simulink model "furuta_harness"  (R2026a)
settings: Solver=ode4  StopTime=hT  FixedStep=hcfg.dt
PostLoadFcn:
  | addpath(fileparts(get_param('furuta_harness', 'FileName')));
  | harness_load('LqrBalance', 'balance', 'IfMissing', true, 'Open', false);
values from neighbouring files (symbols this model uses):
  hp = V.hp    [run_sim.m]
  m = R.metrics    [compare_controllers.m]
  N = round(opts.T/h)    [validate_open_loop.m]
  s = names{code + 1}    [run_sim.m]
  X = xn(n, :)'    [validate_open_loop.m]
undefined symbols (not defined in the file or in its folder): ctrlP, hb, hcfg, hx0, Y, Z
libraries: sm_lib x13, nesl_utility x7
settings Model: Creator=ahmad  LastModifiedBy=ahmad
settings DebuggingCC: AlgebraicLoopMsg=error
settings ExplorerConfigSet: SimMechanicsOpenEditorOnUpdate=off

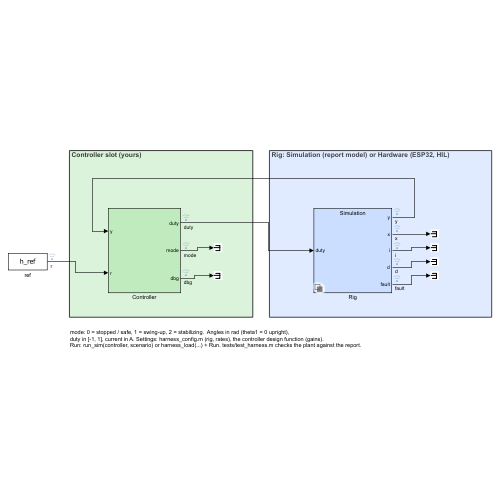
[thumbnail: Simulink's stored preview of the top-level diagram]
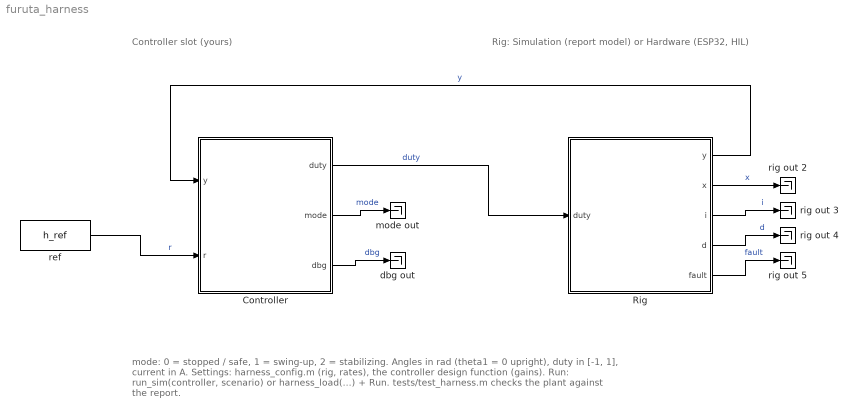
== system furuta_harness ==
  note: Controller slot (yours)
  note: Rig: Simulation (report model) or Hardware (ESP32, HIL)
  note: mode: 0 = stopped / safe, 1 = swing-up, 2 = stabilizing.  Angles in rad (theta1 = 0 upright),
      | duty in [-1, 1], current in A. Settings: harness_config.m (rig, rates), the controller design function (gains).
      | Run: run_sim(controller, scenario) or harness_load(...) + Run. tests/test_harness.m checks the plant against the report.
  Controller : Subsystem
  Rig : Subsystem  Variant=on  VariantControlMode=label  LabelModeActiveChoice=Simulation
  dbg out : Terminator
  mode out : Terminator
  ref : FromWorkspace  VariableName=h_ref  SampleTime=hcfg.Ts  Interpolate=off  OutputAfterFinalValue=Holding final value
  rig out {2..5} (4 alike) : Terminator
  wires:
  ref/1 -> Controller/2(r)  "r"
  Controller/1(duty) -> Rig/1(duty)  "duty"
  Controller/2(mode) -> mode out/1  "mode"
  Controller/3(dbg) -> dbg out/1  "dbg"
  Rig/2(x) -> rig out 2/1  "x"
  Rig/3(i) -> rig out 3/1  "i"
  Rig/4(d) -> rig out 4/1  "d"
  Rig/5(fault) -> rig out 5/1  "fault"
  Rig/1(y) -> Controller/1(y)  "y"

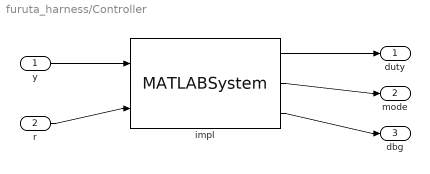
== system furuta_harness/Controller ==
  y : Inport
  r : Inport  Port=2
  impl : MATLABSystem  System=LqrBalance  Ts=hcfg.Ts  P=ctrlP  SimulateUsing=Interpreted execution
      mask Type: LqrBalance
  duty : Outport
  mode : Outport  Port=2
  dbg : Outport  Port=3
  wires:
  y/1 -> impl/1
  r/1 -> impl/2
  impl/1 -> duty/1
  impl/2 -> mode/1
  impl/3 -> dbg/1

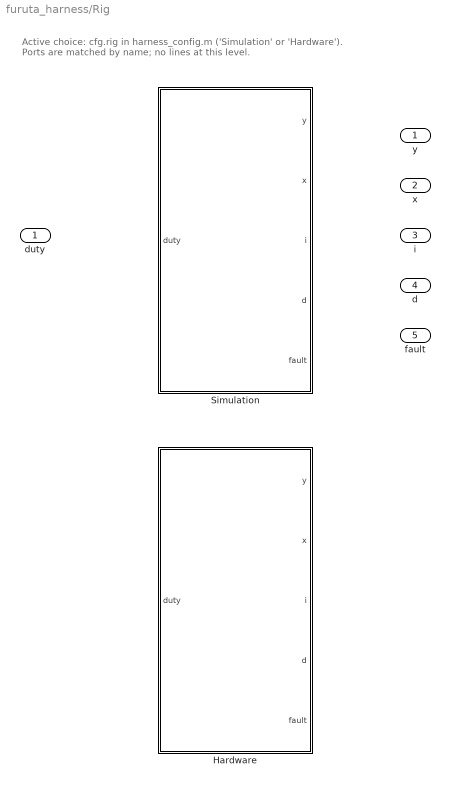
== system furuta_harness/Rig ==
  note: Active choice: cfg.rig in harness_config.m ('Simulation' or 'Hardware').
      | Ports are matched by name; no lines at this level.
  duty : Inport
  Hardware : Subsystem  VariantControl=Hardware
  Simulation : Subsystem  VariantControl=Simulation
  y : Outport
  x : Outport  Port=2
  i : Outport  Port=3
  d : Outport  Port=4
  fault : Outport  Port=5

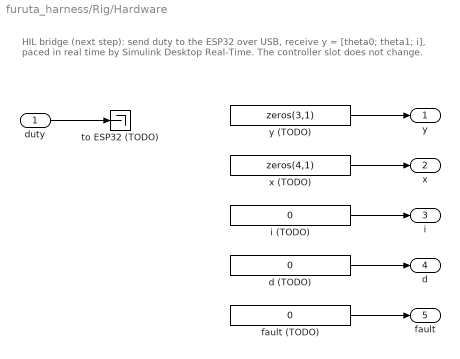
== system furuta_harness/Rig/Hardware ==
  note: HIL bridge (next step): send duty to the ESP32 over USB, receive y = [theta0; theta1; i],
      | paced in real time by Simulink Desktop Real-Time. The controller slot does not change.
  duty : Inport
  d (TODO) : Constant  Value=0  SampleTime=hcfg.Ts
  fault (TODO) : Constant  Value=0  SampleTime=hcfg.Ts
  i (TODO) : Constant  Value=0  SampleTime=hcfg.Ts
  to ESP32 (TODO) : Terminator
  x (TODO) : Constant  Value=zeros(4,1)  SampleTime=hcfg.Ts
  y (TODO) : Constant  Value=zeros(3,1)  SampleTime=hcfg.Ts
  y : Outport
  x : Outport  Port=2
  i : Outport  Port=3
  d : Outport  Port=4
  fault : Outport  Port=5
  wires:
  duty/1 -> to ESP32 (TODO)/1
  y (TODO)/1 -> y/1
  x (TODO)/1 -> x/1
  i (TODO)/1 -> i/1
  d (TODO)/1 -> d/1
  fault (TODO)/1 -> fault/1

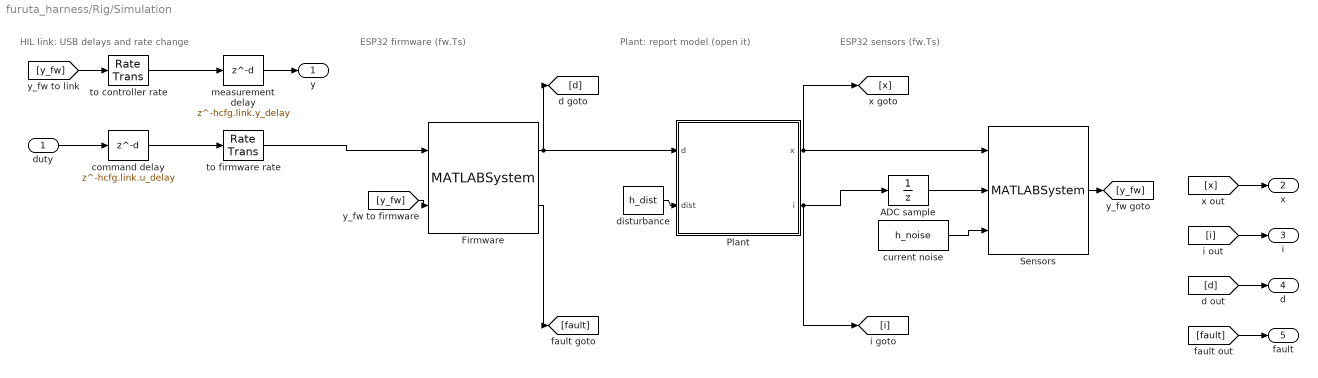
== system furuta_harness/Rig/Simulation ==
  note: HIL link: USB delays and rate change
  note: ESP32 firmware (fw.Ts)
  note: Plant: report model (open it)
  note: ESP32 sensors (fw.Ts)
  duty : Inport
  ADC sample : UnitDelay  SampleTime=hcfg.fw.Ts
  Firmware : MATLABSystem  System=FirmwareActuator  Ts=hcfg.fw.Ts  A=hcfg.act  SimulateUsing=Interpreted execution
      mask Type: FirmwareActuator
  Plant : Subsystem
  Sensors : MATLABSystem  System=FurutaSensors  Ts=hcfg.fw.Ts  S=hcfg.sens  SimulateUsing=Interpreted execution
      mask Type: FurutaSensors
  command delay : Delay  DelayLength=hcfg.link.u_delay  SampleTime=hcfg.Ts
  current noise : FromWorkspace  VariableName=h_noise  SampleTime=hcfg.fw.Ts  Interpolate=off  OutputAfterFinalValue=Holding final value
  disturbance : FromWorkspace  VariableName=h_dist  SampleTime=hcfg.dt  Interpolate=off  OutputAfterFinalValue=Holding final value
  measurement delay : Delay  DelayLength=hcfg.link.y_delay  SampleTime=hcfg.Ts
  to controller rate : RateTransition  Integrity=off  Deterministic=off  OutPortSampleTime=hcfg.Ts
  to firmware rate : RateTransition  Integrity=off  Deterministic=off  OutPortSampleTime=hcfg.fw.Ts
  y : Outport
  x : Outport  Port=2
  i : Outport  Port=3
  d : Outport  Port=4
  fault : Outport  Port=5
  wires:
  [y_fw] -> to controller rate/1
  to controller rate/1 -> measurement delay/1
  measurement delay/1 -> y/1
  duty/1 -> command delay/1
  command delay/1 -> to firmware rate/1
  to firmware rate/1 -> Firmware/1
  [y_fw] -> Firmware/2
  Firmware/2 -> [fault]
  Firmware/1 -> Plant/1(d), [d]
  disturbance/1 -> Plant/2(dist)
  Plant/1(x) -> Sensors/1, [x]
  Plant/2(i) -> ADC sample/1, [i]
  ADC sample/1 -> Sensors/2
  current noise/1 -> Sensors/3
  Sensors/1 -> [y_fw]
  [x] -> x/1
  [i] -> i/1
  [d] -> d/1
  [fault] -> fault/1

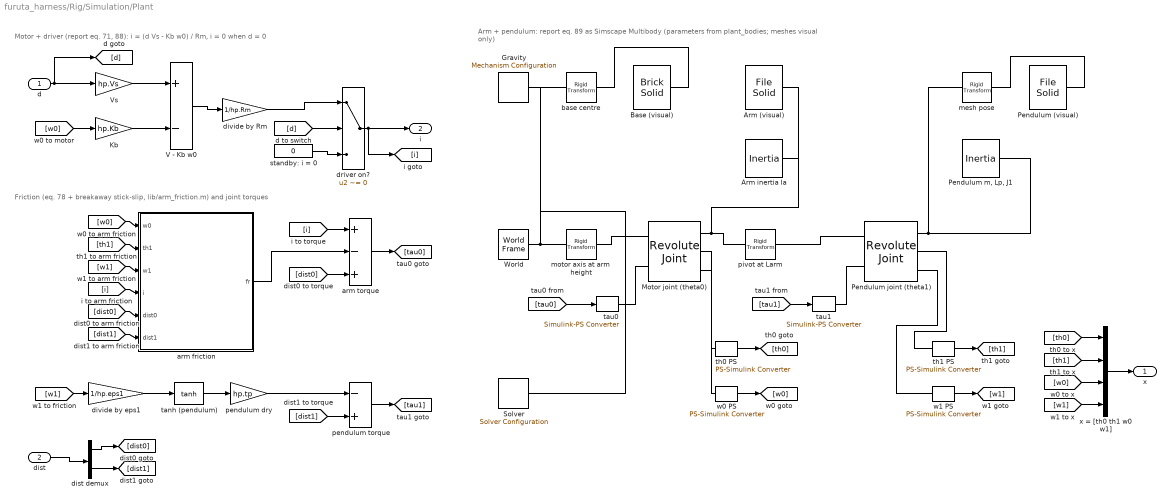
== system furuta_harness/Rig/Simulation/Plant ==
  note: Motor + driver (report eq. 71, 88): i = (d Vs - Kb w0) / Rm, i = 0 when d = 0
  note: Friction (eq. 78 + breakaway stick-slip, lib/arm_friction.m) and joint torques
  note: Arm + pendulum: report eq. 89 as Simscape Multibody (parameters from plant_bodies; meshes visual only)
  d : Inport
  dist : Inport  Port=2
  Arm (visual) : sm_lib/Body Elements/File Solid  ExtGeomFileName=body_arm_jumper3.stl  UnitType=Custom  ExtGeomFileUnits=mm  StepReaderType=HEX  ExportConvexHullGeometry=off  InertiaType=PointMass  BasedOnType=DensityFromFile  Density=1000  DensityUnits=kg/m^3  Mass=1e-9  MassUnits=kg  CenterOfMass=[0 0 0]  CenterOfMassUnits=m  MomentsOfInertia=[1 1 1]  MomentsOfInertiaUnits=kg*m^2  ProductsOfInertia=[0 0 0]  ProductsOfInertiaUnits=kg*m^2  GraphicType=FromGeometry  MarkerShape=Sphere  MarkerSize=10  GraphicVisPropType=SimpleVisualProperties  GraphicDiffuseColor=[0.15 0.15 0.17]  GraphicOpacity=1  GraphicSpecularColor=[0.5 0.5 0.5 1.0]  GraphicAmbientColor=[0.15 0.15 0.15 1.0]  GraphicEmissiveColor=[0.0 0.0 0.0 1.0]  GraphicShininess=75  DoExposeReferenceFrame=on  SerializedFrames=<Frames/>
  Arm inertia Ia : sm_lib/Body Elements/Inertia  InertiaType=Custom  Mass=hb.m_arm  MassUnits=kg  CenterOfMass=[0 0 0]  CenterOfMassUnits=m  MomentsOfInertia=[hb.Ia/2 hb.Ia/2 hb.Ia]  MomentsOfInertiaUnits=kg*m^2  ProductsOfInertia=[0 0 0]  ProductsOfInertiaUnits=kg*m^2  GraphicType=Marker  MarkerShape=Inertia  MarkerSize=20  GraphicVisPropType=SimpleVisualProperties  GraphicDiffuseColor=[0.5 0.5 0.5]  GraphicOpacity=1  GraphicSpecularColor=[0.5 0.5 0.5 1.0]  GraphicAmbientColor=[0.15 0.15 0.15 1.0]  GraphicEmissiveColor=[0.0 0.0 0.0 1.0]  GraphicShininess=75
  Base (visual) : sm_lib/Body Elements/Brick Solid  BrickDimensions=[0.0872 0.0872 0.1]  BrickDimensionsUnits=m  ExportEntireGeometry=off  InertiaType=PointMass  BasedOnType=Density  Density=1000  DensityUnits=kg/m^3  Mass=1e-9  MassUnits=kg  CenterOfMass=[0 0 0]  CenterOfMassUnits=m  MomentsOfInertia=[1 1 1]  MomentsOfInertiaUnits=kg*m^2  ProductsOfInertia=[0 0 0]  ProductsOfInertiaUnits=kg*m^2  GraphicType=FromGeometry  MarkerShape=Sphere  MarkerSize=10  GraphicVisPropType=SimpleVisualProperties  GraphicDiffuseColor=[0.6 0.62 0.65]  GraphicOpacity=0.4  GraphicSpecularColor=[0.5 0.5 0.5 1.0]  GraphicAmbientColor=[0.15 0.15 0.15 1.0]  GraphicEmissiveColor=[0.0 0.0 0.0 1.0]  GraphicShininess=75  DoExposeReferenceFrame=on  SerializedFrames=<Frames/>
  Gravity : sm_lib/Utilities/Mechanism Configuration  UniformGravity=Constant  GravityVector=[0 0 -hb.g]  GravityVectorUnits=m/s^2  LinearizationDelta=0.001  JointModeTransitionNonlinearIterations=2
  Kb : Gain  Gain=hp.Kb
  Motor joint (theta0) : sm_lib/Joints/Revolute Joint  JointMode=Normal  CompositeWrenchDir=FollowerOnBase  CompositeWrenchFrame=BaseFrame  SenseConstraintForce=off  SenseConstraintTorque=off  SenseTotalForce=off  SenseTotalTorque=off  PositionTargetSpecify=on  PositionTargetPriority=High  PositionTargetValue=hx0(1)  PositionTargetValueUnits=rad  VelocityTargetSpecify=on  VelocityTargetPriority=High  VelocityTargetValue=hx0(3)  VelocityTargetValueUnits=rad/s  EquilibriumPosition=0  EquilibriumPositionUnits=deg  SpringStiffness=0  SpringStiffnessUnits=N*m/deg  DampingCoefficient=hp.Beq  DampingCoefficientUnits=N*m/(rad/s)  LowerLimitSpecify=off  LowerLimitBound=-90  LowerLimitBoundUnits=deg  LowerLimitStiffness=1e4  LowerLimitStiffnessUnits=N*m/deg  LowerLimitDamping=10  LowerLimitDampingUnits=N*m/(deg/s)  LowerLimitTransitionRegionWidth=0.1  LowerLimitTransitionRegionWidthUnits=deg  UpperLimitSpecify=off  UpperLimitBound=90  UpperLimitBoundUnits=deg  UpperLimitStiffness=1e4  UpperLimitStiffnessUnits=N*m/deg  UpperLimitDamping=10  UpperLimitDampingUnits=N*m/(deg/s)  UpperLimitTransitionRegionWidth=0.1  UpperLimitTransitionRegionWidthUnits=deg  TorqueActuationMode=InputTorque  MotionActuationMode=ComputedMotion  SensePosition=on  SenseVelocity=on  SenseAcceleration=off  SenseTorqueForce=off  SenseLowerLimitTorqueForce=off  SenseUpperLimitTorqueForce=off
  Pendulum (visual) : sm_lib/Body Elements/File Solid  ExtGeomFileName=body_pendulum_egp.stl  UnitType=Custom  ExtGeomFileUnits=mm  StepReaderType=HEX  ExportConvexHullGeometry=off  InertiaType=PointMass  BasedOnType=DensityFromFile  Density=1000  DensityUnits=kg/m^3  Mass=1e-9  MassUnits=kg  CenterOfMass=[0 0 0]  CenterOfMassUnits=m  MomentsOfInertia=[1 1 1]  MomentsOfInertiaUnits=kg*m^2  ProductsOfInertia=[0 0 0]  ProductsOfInertiaUnits=kg*m^2  GraphicType=FromGeometry  MarkerShape=Sphere  MarkerSize=10  GraphicVisPropType=SimpleVisualProperties  GraphicDiffuseColor=[0.8 0.1 0.1]  GraphicOpacity=1  GraphicSpecularColor=[0.5 0.5 0.5 1.0]  GraphicAmbientColor=[0.15 0.15 0.15 1.0]  GraphicEmissiveColor=[0.0 0.0 0.0 1.0]  GraphicShininess=75  DoExposeReferenceFrame=on  SerializedFrames=<Frames/>
  Pendulum joint (theta1) : sm_lib/Joints/Revolute Joint  JointMode=Normal  CompositeWrenchDir=FollowerOnBase  CompositeWrenchFrame=BaseFrame  SenseConstraintForce=off  SenseConstraintTorque=off  SenseTotalForce=off  SenseTotalTorque=off  PositionTargetSpecify=on  PositionTargetPriority=High  PositionTargetValue=hx0(2)  PositionTargetValueUnits=rad  VelocityTargetSpecify=on  VelocityTargetPriority=High  VelocityTargetValue=hx0(4)  VelocityTargetValueUnits=rad/s  EquilibriumPosition=0  EquilibriumPositionUnits=deg  SpringStiffness=0  SpringStiffnessUnits=N*m/deg  DampingCoefficient=hp.b1  DampingCoefficientUnits=N*m/(rad/s)  LowerLimitSpecify=off  LowerLimitBound=-90  LowerLimitBoundUnits=deg  LowerLimitStiffness=1e4  LowerLimitStiffnessUnits=N*m/deg  LowerLimitDamping=10  LowerLimitDampingUnits=N*m/(deg/s)  LowerLimitTransitionRegionWidth=0.1  LowerLimitTransitionRegionWidthUnits=deg  UpperLimitSpecify=off  UpperLimitBound=90  UpperLimitBoundUnits=deg  UpperLimitStiffness=1e4  UpperLimitStiffnessUnits=N*m/deg  UpperLimitDamping=10  UpperLimitDampingUnits=N*m/(deg/s)  UpperLimitTransitionRegionWidth=0.1  UpperLimitTransitionRegionWidthUnits=deg  TorqueActuationMode=InputTorque  MotionActuationMode=ComputedMotion  SensePosition=on  SenseVelocity=on  SenseAcceleration=off  SenseTorqueForce=off  SenseLowerLimitTorqueForce=off  SenseUpperLimitTorqueForce=off
  "Pendulum m, Lp, J1" : sm_lib/Body Elements/Inertia  InertiaType=Custom  Mass=hb.m  MassUnits=kg  CenterOfMass=[hb.Lp 0 0]  CenterOfMassUnits=m  MomentsOfInertia=[1e-12 hb.J1 hb.J1]  MomentsOfInertiaUnits=kg*m^2  ProductsOfInertia=[0 0 0]  ProductsOfInertiaUnits=kg*m^2  GraphicType=Marker  MarkerShape=Inertia  MarkerSize=20  GraphicVisPropType=SimpleVisualProperties  GraphicDiffuseColor=[0.5 0.5 0.5]  GraphicOpacity=1  GraphicSpecularColor=[0.5 0.5 0.5 1.0]  GraphicAmbientColor=[0.15 0.15 0.15 1.0]  GraphicEmissiveColor=[0.0 0.0 0.0 1.0]  GraphicShininess=75
  Solver : nesl_utility/Solver Configuration  PhysicalDomain=network_engine_domain  SubClassName=solver  LeftPortType=input  RightPortType=generic  Tones=[]  Harmonics=[]  SimulateNoise=off  Profile=off  UseLocalSampling=off  EnableSwitchedLinearOptims=on  FrequencyDomain=off  UseCCode=off  RelTol=0.001  AbsTol=0.001  MinStep=1e-09  ToWorkspace=off  RevertToSquareIcSolve=off  NumHomotopyIterations=100  PhasorMode=off  PhasorModeNumHarmonics=1  ConsistencySolver=NEWTON_XTOL_AFTER_FTOL  CanonicalOrdering=CANONICAL  OptimizeIntermediates=OPTIMIZED  IndexReductionMethod=DerivativeReplacement  DoDC=off  ResidualTolerance=1e-09  ConsistencyTolSource=GLOBAL  ConsistencyAbsTol=0.001  ConsistencyRelTol=0.001  ConsistencyTolFactor=0.001  UseLocalSolver=off  LocalSolverChoice=NE_BACKWARD_EULER_ADVANCER  ResolveIndetEquations=on  FunctionEvalNumThread=1  LocalSolverSampleTime=0.001  DoFixedCost=off  MaxNonlinIter=3  MaxModeIter=2  ComputeImpulses=off  ImpulseIterations=2  LinearAlgebra=auto  LinearAlgebraNumThread=0  EquationFormulation=NE_TIME_EF  DelaysMemoryBudget=1024  AutomaticFiltering=on  FilteringTimeConstant=0.001  PartitionStorageMethod=AS_NEEDED  PartitionMemoryBudget=1024  PartitionMethod=ROBUST  MultibodyUseLocalSolver=off  MultibodyLocalSolverChoice=ODE1  MultibodyLocalSolverSampleTime=0.001
  V - Kb w0 : Sum  Inputs=+-
  Vs : Gain  Gain=hp.Vs
  World : sm_lib/Frames and Transforms/World Frame
  arm friction : MATLAB Function  TreatAsAtomicUnit=on
  arm torque : Sum  Inputs=+-+
  base centre : sm_lib/Frames and Transforms/Rigid Transform  RotationMethod=None  FollAlignAxisA=+X  BaseAlignAxisA=+Y  FollAlignAxisB=+Y  BaseAlignAxisB=+Z  RotationStandardAxis=+Z  RotationAngle=0  RotationAngleUnits=deg  RotationArbitraryAxis=[0 0 1]  RotationSequenceAxes=FollowerAxes  RotationSequence=XYX  RotationSequenceAngles=[0 0 0]  RotationSequenceAnglesUnits=deg  RotationMatrix=[1 0 0;0 1 0;0 0 1]  Quaternion=[1 0 0 0]  TranslationMethod=Cartesian  TranslationCartesianOffset=[0 0 0.05]  TranslationCartesianOffsetUnits=m  TranslationStandardAxis=+Z  TranslationStandardOffset=0  TranslationStandardOffsetUnits=m  TranslationROffset=0  TranslationROffsetUnits=m  TranslationThetaOffset=0  TranslationThetaOffsetUnits=deg  TranslationZOffset=0  TranslationZOffsetUnits=m
  dist demux : Demux  Outputs=2
  divide by Rm : Gain  Gain=1/hp.Rm
  divide by eps1 : Gain  Gain=1/hp.eps1
  driver on? : Switch  Criteria=u2 ~= 0  SaturateOnIntegerOverflow=off  InputSameDT=off
  mesh pose : sm_lib/Frames and Transforms/Rigid Transform  RotationMethod=RotationMatrix  FollAlignAxisA=+X  BaseAlignAxisA=+Y  FollAlignAxisB=+Y  BaseAlignAxisB=+Z  RotationStandardAxis=+Z  RotationAngle=0  RotationAngleUnits=deg  RotationArbitraryAxis=[0 0 1]  RotationSequenceAxes=FollowerAxes  RotationSequence=XYX  RotationSequenceAngles=[0 0 0]  RotationSequenceAnglesUnits=deg  RotationMatrix=[0 0 1; 1 0 0; 0 1 0]  Quaternion=[1 0 0 0]  TranslationMethod=None  TranslationCartesianOffset=[0 0 0]  TranslationCartesianOffsetUnits=m  TranslationStandardAxis=+Z  TranslationStandardOffset=0  TranslationStandardOffsetUnits=m  TranslationROffset=0  TranslationROffsetUnits=m  TranslationThetaOffset=0  TranslationThetaOffsetUnits=deg  TranslationZOffset=0  TranslationZOffsetUnits=m
  motor axis at arm height : sm_lib/Frames and Transforms/Rigid Transform  RotationMethod=None  FollAlignAxisA=+X  BaseAlignAxisA=+Y  FollAlignAxisB=+Y  BaseAlignAxisB=+Z  RotationStandardAxis=+Z  RotationAngle=0  RotationAngleUnits=deg  RotationArbitraryAxis=[0 0 1]  RotationSequenceAxes=FollowerAxes  RotationSequence=XYX  RotationSequenceAngles=[0 0 0]  RotationSequenceAnglesUnits=deg  RotationMatrix=[1 0 0;0 1 0;0 0 1]  Quaternion=[1 0 0 0]  TranslationMethod=Cartesian  TranslationCartesianOffset=[0 0 0.105]  TranslationCartesianOffsetUnits=m  TranslationStandardAxis=+Z  TranslationStandardOffset=0  TranslationStandardOffsetUnits=m  TranslationROffset=0  TranslationROffsetUnits=m  TranslationThetaOffset=0  TranslationThetaOffsetUnits=deg  TranslationZOffset=0  TranslationZOffsetUnits=m
  pendulum dry : Gain  Gain=hp.tp
  pendulum torque : Sum  Inputs=-+
  pivot at Larm : sm_lib/Frames and Transforms/Rigid Transform  RotationMethod=RotationMatrix  FollAlignAxisA=+X  BaseAlignAxisA=+Y  FollAlignAxisB=+Y  BaseAlignAxisB=+Z  RotationStandardAxis=+Z  RotationAngle=0  RotationAngleUnits=deg  RotationArbitraryAxis=[0 0 1]  RotationSequenceAxes=FollowerAxes  RotationSequence=XYX  RotationSequenceAngles=[0 0 0]  RotationSequenceAnglesUnits=deg  RotationMatrix=[0 0 -1; 0 1 0; 1 0 0]  Quaternion=[1 0 0 0]  TranslationMethod=Cartesian  TranslationCartesianOffset=[hb.Larm 0 0.014]  TranslationCartesianOffsetUnits=m  TranslationStandardAxis=+Z  TranslationStandardOffset=0  TranslationStandardOffsetUnits=m  TranslationROffset=0  TranslationROffsetUnits=m  TranslationThetaOffset=0  TranslationThetaOffsetUnits=deg  TranslationZOffset=0  TranslationZOffsetUnits=m
  standby: i = 0 : Constant  Value=0
  tanh (pendulum) : Trigonometry  Operator=tanh
  tau0 : nesl_utility/Simulink-PS Converter  PhysicalDomain=network_engine_domain  SubClassName=ps_input  LeftPortType=input  RightPortType=output  PseudoPeriodic=off  Frequencies=[]  NoiseDistribution=none  NoiseParameters=[]  Unit=N*m  AffineConversion=off  FilteringAndDerivatives=provide  SimscapeFilterOrder=1  InputFilterTimeConstant=0.001  UdotUserProvided=0
  tau1 : nesl_utility/Simulink-PS Converter  PhysicalDomain=network_engine_domain  SubClassName=ps_input  LeftPortType=input  RightPortType=output  PseudoPeriodic=off  Frequencies=[]  NoiseDistribution=none  NoiseParameters=[]  Unit=N*m  AffineConversion=off  FilteringAndDerivatives=provide  SimscapeFilterOrder=1  InputFilterTimeConstant=0.001  UdotUserProvided=0
  th0 PS : nesl_utility/PS-Simulink Converter  PhysicalDomain=network_engine_domain  SubClassName=ps_output  LeftPortType=input  RightPortType=output  PseudoPeriodic=off  Frequencies=[]  VectorFormat=inherit  Unit=rad  AffineConversion=off
  th1 PS : nesl_utility/PS-Simulink Converter  PhysicalDomain=network_engine_domain  SubClassName=ps_output  LeftPortType=input  RightPortType=output  PseudoPeriodic=off  Frequencies=[]  VectorFormat=inherit  Unit=rad  AffineConversion=off
  w0 PS : nesl_utility/PS-Simulink Converter  PhysicalDomain=network_engine_domain  SubClassName=ps_output  LeftPortType=input  RightPortType=output  PseudoPeriodic=off  Frequencies=[]  VectorFormat=inherit  Unit=rad/s  AffineConversion=off
  w1 PS : nesl_utility/PS-Simulink Converter  PhysicalDomain=network_engine_domain  SubClassName=ps_output  LeftPortType=input  RightPortType=output  PseudoPeriodic=off  Frequencies=[]  VectorFormat=inherit  Unit=rad/s  AffineConversion=off
  x = [th0 th1 w0 w1] : Mux
  x : Outport
  i : Outport  Port=2
  wires:
  d/1 -> Vs/1, [d]
  [w0] -> Kb/1
  Vs/1 -> V - Kb w0/1
  Kb/1 -> V - Kb w0/2
  V - Kb w0/1 -> divide by Rm/1
  divide by Rm/1 -> driver on?/1
  [d] -> driver on?/2
  standby: i = 0/1 -> driver on?/3
  driver on?/1 -> i/1, [i]
  [w0] -> arm friction/1(w0)
  [th1] -> arm friction/2(th1)
  [w1] -> arm friction/3(w1)
  [i] -> arm friction/4(i)
  [dist0] -> arm friction/5(dist0)
  [dist1] -> arm friction/6(dist1)
  [w1] -> divide by eps1/1
  divide by eps1/1 -> tanh (pendulum)/1
  tanh (pendulum)/1 -> pendulum dry/1
  dist/1 -> dist demux/1
  dist demux/1 -> [dist0]
  dist demux/2 -> [dist1]
  [i] -> arm torque/1
  arm friction/1(fr) -> arm torque/2
  [dist0] -> arm torque/3
  pendulum dry/1 -> pendulum torque/1
  [dist1] -> pendulum torque/2
  arm torque/1 -> [tau0]
  pendulum torque/1 -> [tau1]
  th0 PS/1 -> [th0]
  w0 PS/1 -> [w0]
  th1 PS/1 -> [th1]
  w1 PS/1 -> [w1]
  [th0] -> x = [th0 th1 w0 w1]/1
  [th1] -> x = [th0 th1 w0 w1]/2
  [w0] -> x = [th0 th1 w0 w1]/3
  [w1] -> x = [th0 th1 w0 w1]/4
  x = [th0 th1 w0 w1]/1 -> x/1
  [tau0] -> tau0/1
  [tau1] -> tau1/1
  connections:
  Motor joint (theta0)/RConn2 -- th0 PS/LConn1
  Motor joint (theta0)/RConn3 -- w0 PS/LConn1
  Pendulum joint (theta1)/RConn2 -- th1 PS/LConn1
  Pendulum joint (theta1)/RConn3 -- w1 PS/LConn1
  Gravity/RConn1 -- World/RConn1 -- Solver/RConn1 -- base centre/LConn1 -- motor axis at arm height/LConn1
  base centre/RConn1 -- Base (visual)/RConn1
  motor axis at arm height/RConn1 -- Motor joint (theta0)/LConn1
  tau0/RConn1 -- Motor joint (theta0)/LConn2
  pivot at Larm/LConn1 -- Motor joint (theta0)/RConn1 -- Arm inertia Ia/RConn1 -- Arm (visual)/RConn1
  pivot at Larm/RConn1 -- Pendulum joint (theta1)/LConn1
  tau1/RConn1 -- Pendulum joint (theta1)/LConn2
  "Pendulum m, Lp, J1"/RConn1 -- Pendulum joint (theta1)/RConn1 -- mesh pose/LConn1
  mesh pose/RConn1 -- Pendulum (visual)/RConn1

== matlab function furuta_harness/Rig/Simulation/Plant/arm friction ==
  data: w0 input; fr output; th1 input; w1 input; i input; dist0 input; dist1 input; hp parameter
function fr = arm_dry_friction(w0, th1, w1, i, dist0, dist1, hp)
% Arm dry friction [A]: sliding Coulomb + breakaway stick-slip (lib/arm_friction.m, = furuta_rhs).
fr = arm_friction(w0, th1, w1, i, [dist0; dist1], hp);
